simulink model "ASM_Traffic"  (R2026a)
settings: Solver=ode1  StartTime=SIM.tstart.v  StopTime=SIM.tend.v  FixedStep=SIM.StepSize.v
PostLoadFcn:
  | if any(exist('dsrtsu_mdlpostloadfcn', 'file') ~= 0), dsrtsu_mdlpostloadfcn('Execute', bdroot); end
  | try, asm_mdl_postloadfcn(bdroot, 'UpdateModel', 3600); catch, disp(lasterr); end,
InitFcn:
  | , if any(exist('rtifpga_mdlclblib', 'file') ~= 0), rtifpga_mdlclblib('Init', bdroot); end,
  | , if any(exist('dsmpb_private', 'file') ~= 0), dsmpb_private('dsmpb_mdlclblib', 'Init', bdroot); end,
model workspace (MAT data in the model file):
  asmReferencePath = [0 0.01 0.02 0.03 0.04 0.05 0.06 0.07 0.08 0.09 0.1 0.11 ... (350007 elements, 50001x7)]
  roadBounds : Simulink.Parameter (value not decoded)
  safetyAxes : Simulink.Parameter (value not decoded)
undefined symbols (not defined in the file): _to_, a0b2, ASM_BrakeHydraulics_DemoSystems, ASM_VehicleDynamics_DemoSystems, b98103fe8ad365046cd0, BrakeCircuit, controllerConfig, CPT, Crankshaft, DiscIntNeverNeededParam, dsmsi, FinalDriveAssembly, MDL, ModeSignals, mu, Pos_BrakePedal_Maneuver, rad, RefSignals, roadFamilyData, roadFamilyId, s_to_rpm, SIM, SoftECU, Suspension, Tire, Transmission
libraries: ASM_Traffic_lib x135, simulink x98, ASM_Utils_lib x77, ASM_VehicleDynamics_lib x70, ASM_Environment_lib x22, dsmpblib x20, dsmsilib x15, MDLD_Utils_lib x10, ASM_BrakeHydraulics_lib x3, sl_discontinuities x2
(part 33 of 65)

== system ASM_Traffic/VehicleDynamics/Plant/VehicleDynamics/TireMapping_CP ==
  Sw_Tire_Parameter_Set_CP[:][1|2|3|4] : Inport
  Fric_Coeff_CP[:][] : Inport  Port=2
  Pos_z_CP[:][m] : Inport  Port=3
  UnitVec_z_CP[:][x;y;z] : Inport  Port=4
  Selector : Selector  IndexOptions=Index vector (dialog)  Indices=[1:4]  OutputSizes=1
  Selector1 : Selector  IndexOptions=Index vector (dialog)  Indices=[1:4]  OutputSizes=1
  Selector2 : Selector  IndexOptions=Index vector (dialog)  Indices=[1:4]  OutputSizes=1
  Selector3 : Selector  IndexOptions=Index vector (dialog)  Indices=[1:12]  OutputSizes=1
  Sw_Tire_Parameter_Set_CP_Veh[FL;FR;RL;RR][1|2|3|4] : Outport  VectorParamsAs1DForOutWhenUnconnected=off
  Fric_Coeff_CP_Veh[FL;FR;RL;RR][] : Outport  Port=2  VectorParamsAs1DForOutWhenUnconnected=off
  Pos_z_CP_Veh[FL;FR;RL;RR][m] : Outport  Port=3  VectorParamsAs1DForOutWhenUnconnected=off
  UnitVec_z_CP_Veh[FL;FR;RL;RR][x;y;z] : Outport  Port=4  VectorParamsAs1DForOutWhenUnconnected=off
  wires:
  Selector2/1 -> Sw_Tire_Parameter_Set_CP_Veh[FL;FR;RL;RR][1|2|3|4]/1
  Selector3/1 -> UnitVec_z_CP_Veh[FL;FR;RL;RR][x;y;z]/1
  Selector1/1 -> Fric_Coeff_CP_Veh[FL;FR;RL;RR][]/1
  Selector/1 -> Pos_z_CP_Veh[FL;FR;RL;RR][m]/1
  Pos_z_CP[:][m]/1 -> Selector/1
  Fric_Coeff_CP[:][]/1 -> Selector1/1
  UnitVec_z_CP[:][x;y;z]/1 -> Selector3/1
  Sw_Tire_Parameter_Set_CP[:][1|2|3|4]/1 -> Selector2/1

== system ASM_Traffic/VehicleDynamics/Plant/VehicleDynamics/VehicleInits ==
  q_dt_Vehicle_Init[6x1] : Inport
  q_dt_Wheel_Init[:] : Inport  Port=2
  q_Wheel_Init_In[:] : Inport  Port=3
  Bus Selector : BusSelector  OutputSignals=Tire_allSignals.Tire_FL.Tire.r_Dyn_Tire[m],Tire_allSignals.Tire_FR.Tire.r_Dyn_Tire[m],Tire_allSignals.Tire_RL.Tire.r_Dyn_Tire[m],Tire_allSignals.Tire_RR.Tire.r_Dyn_Tire[m]
  Mux : Mux  Inputs=2
  Mux1 : Mux
  Product : Product  Inputs=/*  RndMeth=Zero
  Saturation : Saturate  UpperLimit=inf  LowerLimit=0.01
  Unit Delay : UnitDelay  SampleTime=-1
  v_x_Init[m|s] : Selector  InputPortWidth=6  IndexOptions=Index vector (dialog)  Indices=[1]  OutputSizes=1
  omega_Wheel_Init[:][rad|s] : Outport  VectorParamsAs1DForOutWhenUnconnected=off
  q_dt_Init[:] : Outport  Port=2  VectorParamsAs1DForOutWhenUnconnected=off
  q_Wheel_Init[:] : Outport  Port=3  VectorParamsAs1DForOutWhenUnconnected=off
  wires:
  q_dt_Vehicle_Init[6x1]/1 -> v_x_Init[m|s]/1, Mux/1
  Mux1/1 -> Saturation/1
  Bus Selector/4 -> Mux1/4  "<r_Dyn_Tire[m]>"
  Bus Selector/3 -> Mux1/3  "<r_Dyn_Tire[m]>"
  Bus Selector/2 -> Mux1/2  "<r_Dyn_Tire[m]>"
  v_x_Init[m|s]/1 -> Product/2
  Mux/1 -> q_dt_Init[:]/1
  q_Wheel_Init_In[:]/1 -> q_Wheel_Init[:]/1
  q_dt_Wheel_Init[:]/1 -> Mux/2
  Saturation/1 -> Product/1
  Bus Selector/1 -> Mux1/1  "<r_Dyn_Tire[m]>"
  Unit Delay/1 -> omega_Wheel_Init[:][rad|s]/1
  Product/1 -> Unit Delay/1
  [ASMBUS_VehicleDynamics_Tire] -> Bus Selector/1

== system ASM_Traffic/VehicleDynamics/Plant/VehicleDynamics/VehicleMovement ==
  F_Aero_CoorSys_V[x;y;z][N] : Inport
  Trq_Aero_CoorSys_V[x;y;z][Nm] : Inport  Port=2
  F_Tire_CoorSys_V[FL,FR,RL,RR][x;y;z][N] : Inport  Port=3
  Trq_Tire_CoorSys_V[FL,FR,RL,RR][x;y;z][Nm] : Inport  Port=4
  Stiffness_z_Tire[FL,FR,RL,RR][N|m] : Inport  Port=5
  w_Wheel[FL,FR,RL,RR][x;y;z][rad|s] : Inport  Port=6
  Trq_Shaft_CoorSys_V[FL,FR,RL,RR][x;y;z][Nm] : Inport  Port=7
  gF_Susp[q1_Front;q2_Front;q1_Rear;q2_Rear][] : Inport  Port=8
  Pos_Wheel[FL,FR,RL,RR][x;y;z][m] : Inport  Port=9
  w_Rel_WheelBody[FL,FR,RL,RR][x y z][rad|s] : Inport  Port=10
  v_Rel_WheelBody[FL,FR,RL,RR][x;y;z][m|s] : Inport  Port=11
  Pos_Vehicle_Init_CoorSys_E[x;y;z][m] : Inport  Port=12
  Angle_V_Init_CoorSys_E[x;y;z][rad] : Inport  Port=13
  Reset[] : Inport  Port=14
  KeepVehiclePosition[0|1] : Inport  Port=15
  gRear_dq_Rear_dt[2x2][] : Inport  Port=16
  gFront_dq_Front_dt[2x2][] : Inport  Port=17
  SuspensionKinematicsRelations_Rear : Inport  Port=18
  SuspensionKinematicsRelations_Front : Inport  Port=19
  F_External_CoorSys_V[x,y,z][N] : Inport  Port=20
  Trq_External_CoorSys_V[x,y,z][Nm] : Inport  Port=21
  Stabilization_F_External[3X6] : Inport  Port=22
  Stabilization_Trq_External[3X6] : Inport  Port=23
  q_dt_Init[:] : Inport  Port=24
  q_Wheel_Init[:] : Inport  Port=25
  ASMSignalCollector : Subsystem
  Bus Selector1 : BusSelector  OutputSignals=Pos_RL_Wheel_dq_Rear[q1;q2][x;y;z][],w_Rel_RL_Wheel_dq_Rear_dt[q1;q2][x;y;z][],Pos_RR_Wheel_dq_Rear[q1;q2][x;y;z][],w_Rel_RR_Wheel_dq_Rear[q1;q2][x;y;z][]
  Bus Selector2 : BusSelector  OutputSignals=Pos_FL_Wheel_dq_Front[q1;q2][x;y;z][],w_Rel_FL_Wheel_dq_Front_dt[q1;q2][x;y;z][],Pos_FR_Wheel_dq_Front[q1;q2][x;y;z][],w_Rel_FR_Wheel_dq_Front[q1;q2][x;y;z][]
  COORDINATE_TRANSFORMATION : ASM_VehicleDynamics_lib/VehicleDynamics/VehicleMovement/COORDINATE_TRANSFORMATION  Tag=ASM_SUBCOMPONENT  StepSize=SIM.StepSize  ASMProperties=struct('Name','COORDINATE_TRANSFORMATION','Version','5.0','Library','ASM_VehicleDynamics_lib')  ASMInstanceName=coordinate_transformation  ASMInstanceID=1
  Goto Tag Visibility : GotoTagVisibility  GotoTag=ASMBUS_VehicleDynamics_VehicleMotion
  Goto Tag Visibility1 : GotoTagVisibility  GotoTag=ASMBUS_VehicleDynamics_CoGAndWheelVelocities
  Goto Tag Visibility2 : GotoTagVisibility  GotoTag=ASMBUS_VehicleDynamics_SensorMotion
  Goto Tag Visibility3 : GotoTagVisibility  GotoTag=ASMBUS_VehicleDynamics_MassForcesAndTorques
  Goto Tag Visibility4 : GotoTagVisibility  GotoTag=ASMBUS_VehicleDynamics_CoordinateTransformation
  Goto Tag Visibility5 : GotoTagVisibility  GotoTag=ASMBUS_VehicleDynamics_VehicleMass
  J : Constant  Value=zeros(3,3)
  MASS_FORCES_AND_TORQUES : ASM_VehicleDynamics_lib/VehicleDynamics/VehicleMovement/MASS_FORCES_AND_TORQUES  Tag=ASM_SUBCOMPONENT  ASMProperties=struct('Name','MASS_FORCES_AND_TORQUES','Version','3.0','Library','ASM_VehicleDynamics_lib')  ASMInstanceName=mass_forces_and_torques  ASMInstanceID=1
  OR : Subsystem
  SENSOR_MOTION : ASM_VehicleDynamics_lib/VehicleDynamics/VehicleMovement/SENSOR_MOTION  Tag=ASM_SUBCOMPONENT  Const_PosVec_Sensor1=MDL.VehicleDynamics.VehicleMovement.SensorMotion.Const_PosVec_Sensor1  Const_PosVec_Sensor2=MDL.VehicleDynamics.VehicleMovement.SensorMotion.Const_PosVec_Sensor2  Const_PosVec_Sensor3=MDL.VehicleDynamics.VehicleMovement.SensorMotion.Const_PosVec_Sensor3  Const_PosVec_Sensor4=MDL.VehicleDynamics.VehicleMovement.SensorMotion.Const_PosVec_Sensor4  ASMProperties=struct('Name','SENSOR_MOTION','Version','5.0','Library','ASM_VehicleDynamics_lib')  ASMInstanceName=sensor_motion  ASMInstanceID=1
  Selector1 : Selector  InputPortWidth=15  IndexOptions=Index vector (dialog)  Indices=[4:15]  OutputSizes=1
  Selector2 : Selector  InputPortWidth=15  IndexOptions=Index vector (dialog)  Indices=[4:15]  OutputSizes=1
  Selector3 : Selector  InputPortWidth=15  IndexOptions=Index vector (dialog)  Indices=[4:15]  OutputSizes=1
  Sw_TestBenchMode[1Vehicle|2TestBench] : Constant
  Terminator : Terminator
  VEHICLE_AND_WHEEL_VELOCITIES : ASM_VehicleDynamics_lib/VehicleDynamics/VehicleMovement/VEHICLE_AND_WHEEL_VELOCITIES  Tag=ASM_SUBCOMPONENT  ASMProperties=struct('Name','VEHICLE_AND_WHEEL_VELOCITIES','Version','1.0','Library','ASM_VehicleDynamics_lib')  ASMInstanceName=vehicle_and_wheel_velocities  ASMInstanceID=1
  VEHICLE_MASS_AND_ADDITIONAL_LOADS : ASM_VehicleDynamics_lib/VehicleDynamics/VehicleMovement/VEHICLE_MASS_AND_ADDITIONAL_LOADS  Tag=ASM_SUBCOMPONENT  Const_m_Vehicle=MDL.VehicleDynamics.Vehicle.Const_m_Vehicle  Const_PosVec_CoG_Vehicle=MDL.VehicleDynamics.Vehicle.Const_PosVec_CoG_Vehicle  Const_Inertia_Tensor_Vehicle=MDL.VehicleDynamics.Vehicle.Const_Inertia_Tensor_Vehicle  Const_m_AddLoad1=MDL.VehicleDynamics.VehicleMovement.AddLoad1.Const_m_AddLoad1  Const_PosVec_CoG_AddLoad1=MDL.VehicleDynamics.VehicleMovement.AddLoad1.Const_PosVec_CoG_AddLoad1  Const_Inertia_Tensor_AddLoad1=MDL.VehicleDynamics.VehicleMovement.AddLoad1.Const_Inertia_Tensor_AddLoad1  Sw_AddLoad1=MDL.VehicleDynamics.VehicleMovement.AddLoad1.Sw_AddLoad1  Const_m_AddLoad2=MDL.VehicleDynamics.VehicleMovement.AddLoad2.Const_m_AddLoad2  Const_PosVec_CoG_AddLoad2=MDL.VehicleDynamics.VehicleMovement.AddLoad2.Const_PosVec_CoG_AddLoad2  Const_Inertia_Tensor_AddLoad2=MDL.VehicleDynamics.VehicleMovement.AddLoad2.Const_Inertia_Tensor_AddLoad2  Sw_AddLoad2=MDL.VehicleDynamics.VehicleMovement.AddLoad2.Sw_AddLoad2  Const_m_AddLoad3=MDL.VehicleDynamics.VehicleMovement.AddLoad3.Const_m_AddLoad3  Const_PosVec_CoG_AddLoad3=MDL.VehicleDynamics.VehicleMovement.AddLoad3.Const_PosVec_CoG_AddLoad3  Const_Inertia_Tensor_AddLoad3=MDL.VehicleDynamics.VehicleMovement.AddLoad3.Const_Inertia_Tensor_AddLoad3  Sw_AddLoad3=MDL.VehicleDynamics.VehicleMovement.AddLoad3.Sw_AddLoad3  Const_m_AddLoad4=MDL.VehicleDynamics.VehicleMovement.AddLoad4.Const_m_AddLoad4  Const_PosVec_CoG_AddLoad4=MDL.VehicleDynamics.VehicleMovement.AddLoad4.Const_PosVec_CoG_AddLoad4  Const_Inertia_Tensor_AddLoad4=MDL.VehicleDynamics.VehicleMovement.AddLoad4.Const_Inertia_Tensor_AddLoad4  Sw_AddLoad4=MDL.VehicleDynamics.VehicleMovement.AddLoad4.Sw_AddLoad4  Const_m_AddLoad5=MDL.VehicleDynamics.VehicleMovement.AddLoad5.Const_m_AddLoad5  Const_PosVec_CoG_AddLoad5=MDL.VehicleDynamics.VehicleMovement.AddLoad5.Const_PosVec_CoG_AddLoad5  Const_Inertia_Tensor_AddLoad5=MDL.VehicleDynamics.VehicleMovement.AddLoad5.Const_Inertia_Tensor_AddLoad5  Sw_AddLoad5=MDL.VehicleDynamics.VehicleMovement.AddLoad5.Sw_AddLoad5  Const_m_AddLoad6=MDL.VehicleDynamics.VehicleMovement.AddLoad6.Const_m_AddLoad6  Const_PosVec_CoG_AddLoad6=MDL.VehicleDynamics.VehicleMovement.AddLoad6.Const_PosVec_CoG_AddLoad6  Const_Inertia_Tensor_AddLoad6=MDL.VehicleDynamics.VehicleMovement.AddLoad6.Const_Inertia_Tensor_AddLoad6  Sw_AddLoad6=MDL.VehicleDynamics.VehicleMovement.AddLoad6.Sw_AddLoad6  ASMProperties=struct('Name','VEHICLE_MASS_AND_ADDITIONAL_LOADS','Version','4.0','Library','ASM_VehicleDynamics_lib')  ASMInstanceName=vehicle_mass_and_additional_loads  ASMInstanceID=1
  VEHICLE_MOTION_CAR : ASM_VehicleDynamics_lib/VehicleDynamics/VehicleMovement/VEHICLE_MOTION_CAR  Tag=ASM_SUBCOMPONENT  StepSize=SIM.StepSize  ASMProperties=struct('Name','VEHICLE_MOTION_CAR','Version','6.0','Library','ASM_VehicleDynamics_lib')  ASMInstanceName=vehicle_motion_car  ASMInstanceID=1
  m : Constant  Value=0
  r_CoG : Constant  Value=[0 0 0]
  ASMSignalBus : Outport  VectorParamsAs1DForOutWhenUnconnected=off
  v_Abs_Vehicle_CoG[x;y;z][m|s] : Outport  Port=2  VectorParamsAs1DForOutWhenUnconnected=off
  RotationMatrix_V_to_E_T[3x3] : Outport  Port=3  VectorParamsAs1DForOutWhenUnconnected=off
  Pos_Wheels_CoorSys_E[FL,FR,RL,RR][x;y;z][m] : Outport  Port=4  VectorParamsAs1DForOutWhenUnconnected=off
  v_Abs_WheelBody_CoorSys_V[FL,FR,RL,RR][x y z][m|s] : Outport  Port=5  VectorParamsAs1DForOutWhenUnconnected=off
  w_Abs_Wheel_CoorSys_V[FL,FR,RL,RR][x,y,z][rad|s] : Outport  Port=6  VectorParamsAs1DForOutWhenUnconnected=off
  F_Gyroscopic[FL,FR,RL,RR][x;y;z][N] : Outport  Port=7  VectorParamsAs1DForOutWhenUnconnected=off
  Trq_Gyroscopic[FL,FR,RL,RR][x;y;z][Nm] : Outport  Port=8  VectorParamsAs1DForOutWhenUnconnected=off
  F_Gravitational[FL,FR,RL,RR][x;y;z][N] : Outport  Port=9  VectorParamsAs1DForOutWhenUnconnected=off
  q_Wheel_dt[q1_Front;q2_Front;q1_Rear;q2_Rear][] : Outport  Port=10  VectorParamsAs1DForOutWhenUnconnected=off
  q_Wheel[q1_Front;q2_Front;q1_Rear;q2_Rear][] : Outport  Port=11  VectorParamsAs1DForOutWhenUnconnected=off
  tag scope: ASMBUS_VehicleDynamics_CoGAndWheelVelocities=scoped, ASMBUS_VehicleDynamics_CoordinateTransformation=scoped, ASMBUS_VehicleDynamics_MassForcesAndTorques=scoped, ASMBUS_VehicleDynamics_SensorMotion=scoped, ASMBUS_VehicleDynamics_VehicleMass=global, ASMBUS_VehicleDynamics_VehicleMotion=scoped
  wires:
  COORDINATE_TRANSFORMATION/1 -> [ASMBUS_VehicleDynamics_CoordinateTransformation]
  VEHICLE_AND_WHEEL_VELOCITIES/1 -> [ASMBUS_VehicleDynamics_CoGAndWheelVelocities]
  VEHICLE_MOTION_CAR/1 -> [ASMBUS_VehicleDynamics_VehicleMotion]
  VEHICLE_AND_WHEEL_VELOCITIES/3 -> w_Abs_Wheel_CoorSys_V[FL,FR,RL,RR][x,y,z][rad|s]/1
  VEHICLE_AND_WHEEL_VELOCITIES/5 -> MASS_FORCES_AND_TORQUES/2, v_Abs_Vehicle_CoG[x;y;z][m|s]/1
  VEHICLE_AND_WHEEL_VELOCITIES/4 -> MASS_FORCES_AND_TORQUES/1, v_Abs_WheelBody_CoorSys_V[FL,FR,RL,RR][x y z][m|s]/1
  VEHICLE_AND_WHEEL_VELOCITIES/6 -> MASS_FORCES_AND_TORQUES/3
  MASS_FORCES_AND_TORQUES/3 -> Selector1/1, VEHICLE_MOTION_CAR/14
  MASS_FORCES_AND_TORQUES/2 -> Selector2/1, VEHICLE_MOTION_CAR/15
  VEHICLE_MOTION_CAR/6 -> VEHICLE_AND_WHEEL_VELOCITIES/2, MASS_FORCES_AND_TORQUES/4, COORDINATE_TRANSFORMATION/4, SENSOR_MOTION/4
  VEHICLE_MOTION_CAR/7 -> COORDINATE_TRANSFORMATION/3, SENSOR_MOTION/3, VEHICLE_AND_WHEEL_VELOCITIES/1
  MASS_FORCES_AND_TORQUES/1 -> [ASMBUS_VehicleDynamics_MassForcesAndTorques]
  VEHICLE_MASS_AND_ADDITIONAL_LOADS/1 -> [ASMBUS_VehicleDynamics_VehicleMass]
  VEHICLE_MASS_AND_ADDITIONAL_LOADS/4 -> VEHICLE_AND_WHEEL_VELOCITIES/7, VEHICLE_MOTION_CAR/10
  VEHICLE_MASS_AND_ADDITIONAL_LOADS/3 -> MASS_FORCES_AND_TORQUES/9, VEHICLE_MOTION_CAR/11
  VEHICLE_MASS_AND_ADDITIONAL_LOADS/2 -> MASS_FORCES_AND_TORQUES/8, VEHICLE_MOTION_CAR/12
  VEHICLE_MOTION_CAR/2 -> q_Wheel_dt[q1_Front;q2_Front;q1_Rear;q2_Rear][]/1
  w_Rel_WheelBody[FL,FR,RL,RR][x y z][rad|s]/1 -> VEHICLE_AND_WHEEL_VELOCITIES/5
  v_Rel_WheelBody[FL,FR,RL,RR][x;y;z][m|s]/1 -> MASS_FORCES_AND_TORQUES/5, VEHICLE_AND_WHEEL_VELOCITIES/4
  w_Wheel[FL,FR,RL,RR][x;y;z][rad|s]/1 -> MASS_FORCES_AND_TORQUES/6, VEHICLE_AND_WHEEL_VELOCITIES/6
  VEHICLE_MOTION_CAR/4 -> SENSOR_MOTION/1
  VEHICLE_MOTION_CAR/5 -> SENSOR_MOTION/2
  SENSOR_MOTION/1 -> [ASMBUS_VehicleDynamics_SensorMotion]
  MASS_FORCES_AND_TORQUES/4 -> Selector3/1, VEHICLE_MOTION_CAR/13
  VEHICLE_AND_WHEEL_VELOCITIES/2 -> Terminator/1
  COORDINATE_TRANSFORMATION/2 -> Pos_Wheels_CoorSys_E[FL,FR,RL,RR][x;y;z][m]/1
  COORDINATE_TRANSFORMATION/3 -> RotationMatrix_V_to_E_T[3x3]/1
  Pos_Vehicle_Init_CoorSys_E[x;y;z][m]/1 -> COORDINATE_TRANSFORMATION/5
  Angle_V_Init_CoorSys_E[x;y;z][rad]/1 -> COORDINATE_TRANSFORMATION/6
  COORDINATE_TRANSFORMATION/4 -> MASS_FORCES_AND_TORQUES/7, SENSOR_MOTION/5
  VEHICLE_MOTION_CAR/3 -> q_Wheel[q1_Front;q2_Front;q1_Rear;q2_Rear][]/1
  Reset[]/1 -> ASMSignalCollector/1(Reset[]), COORDINATE_TRANSFORMATION/1, OR/2(In2)
  gF_Susp[q1_Front;q2_Front;q1_Rear;q2_Rear][]/1 -> VEHICLE_MOTION_CAR/2
  Pos_Wheel[FL,FR,RL,RR][x;y;z][m]/1 -> COORDINATE_TRANSFORMATION/2, VEHICLE_AND_WHEEL_VELOCITIES/3, VEHICLE_MOTION_CAR/3
  F_Tire_CoorSys_V[FL,FR,RL,RR][x;y;z][N]/1 -> VEHICLE_MOTION_CAR/4
  Trq_Tire_CoorSys_V[FL,FR,RL,RR][x;y;z][Nm]/1 -> VEHICLE_MOTION_CAR/5
  F_Aero_CoorSys_V[x;y;z][N]/1 -> VEHICLE_MOTION_CAR/6
  Trq_Aero_CoorSys_V[x;y;z][Nm]/1 -> VEHICLE_MOTION_CAR/7
  Stiffness_z_Tire[FL,FR,RL,RR][N|m]/1 -> VEHICLE_MOTION_CAR/8
  Trq_Shaft_CoorSys_V[FL,FR,RL,RR][x;y;z][Nm]/1 -> VEHICLE_MOTION_CAR/9
  gFront_dq_Front_dt[2x2][]/1 -> VEHICLE_MOTION_CAR/24
  gRear_dq_Rear_dt[2x2][]/1 -> VEHICLE_MOTION_CAR/25
  SuspensionKinematicsRelations_Front/1 -> Bus Selector2/1
  Bus Selector2/1 -> VEHICLE_MOTION_CAR/16  "<Pos_FL_Wheel_dq_Front[q1;q2][x;y;z][]>"
  Bus Selector2/2 -> VEHICLE_MOTION_CAR/17  "<w_Rel_FL_Wheel_dq_Front_dt[q1;q2][x;y;z][]>"
  Bus Selector2/3 -> VEHICLE_MOTION_CAR/18  "<Pos_FR_Wheel_dq_Front[q1;q2][x;y;z][]>"
  Bus Selector2/4 -> VEHICLE_MOTION_CAR/19  "<w_Rel_FR_Wheel_dq_Front[q1;q2][x;y;z][]>"
  Bus Selector1/1 -> VEHICLE_MOTION_CAR/20  "<Pos_RL_Wheel_dq_Rear[q1;q2][x;y;z][]>"
  Bus Selector1/2 -> VEHICLE_MOTION_CAR/21  "<w_Rel_RL_Wheel_dq_Rear_dt[q1;q2][x;y;z][]>"
  Bus Selector1/3 -> VEHICLE_MOTION_CAR/22  "<Pos_RR_Wheel_dq_Rear[q1;q2][x;y;z][]>"
  Bus Selector1/4 -> VEHICLE_MOTION_CAR/23  "<w_Rel_RR_Wheel_dq_Rear[q1;q2][x;y;z][]>"
  SuspensionKinematicsRelations_Rear/1 -> Bus Selector1/1
  ASMSignalCollector/1(ASMSignalBus) -> ASMSignalBus/1
  Selector2/1 -> Trq_Gyroscopic[FL,FR,RL,RR][x;y;z][Nm]/1
  Selector1/1 -> F_Gyroscopic[FL,FR,RL,RR][x;y;z][N]/1
  Selector3/1 -> F_Gravitational[FL,FR,RL,RR][x;y;z][N]/1
  F_External_CoorSys_V[x,y,z][N]/1 -> VEHICLE_MOTION_CAR/26
  Trq_External_CoorSys_V[x,y,z][Nm]/1 -> VEHICLE_MOTION_CAR/27
  Stabilization_F_External[3X6]/1 -> VEHICLE_MOTION_CAR/28
  Stabilization_Trq_External[3X6]/1 -> VEHICLE_MOTION_CAR/29
  Sw_TestBenchMode[1Vehicle|2TestBench]/1 -> VEHICLE_MOTION_CAR/30
  KeepVehiclePosition[0|1]/1 -> OR/1(In1)
  OR/1(Out) -> VEHICLE_MOTION_CAR/1
  q_dt_Init[:]/1 -> VEHICLE_MOTION_CAR/31
  q_Wheel_Init[:]/1 -> VEHICLE_MOTION_CAR/32
  COORDINATE_TRANSFORMATION/5 -> SENSOR_MOTION/6
  J/1 -> VEHICLE_MASS_AND_ADDITIONAL_LOADS/3
  r_CoG/1 -> VEHICLE_MASS_AND_ADDITIONAL_LOADS/2
  m/1 -> VEHICLE_MASS_AND_ADDITIONAL_LOADS/1

== system ASM_Traffic/VehicleDynamics/Plant/VehicleDynamics/avoid_incomplete_trace2source ==
  In1 : Inport
  DummyGain : Gain
  Out1 : Outport
  wires:
  DummyGain/1 -> Out1/1
  In1/1 -> DummyGain/1

== system ASM_Traffic/VehicleDynamics/Plant/VehicleDynamics/avoid_incomplete_trace2source1 ==
  In1 : Inport
  DummyGain : Gain
  Out1 : Outport
  wires:
  DummyGain/1 -> Out1/1
  In1/1 -> DummyGain/1

== system ASM_Traffic/VehicleDynamics/Plant/VehicleDynamics/avoid_incomplete_trace2source2 ==
  In1 : Inport
  DummyGain : Gain
  Out1 : Outport
  wires:
  DummyGain/1 -> Out1/1
  In1/1 -> DummyGain/1
